simulink model "model_new"  (R2023a)
settings: Solver=VariableStepAuto  StartTime=0.0  StopTime=0.5  RelTol=1e-3
model workspace: external: MATLAB File model_new_DataFile.m (data not in the file)
values from neighbouring files (symbols this model uses):
  smiData = struct    [model_new_DataFile.m]
undefined symbols (not defined in the file or in its folder): _, ____, ____16, ____19, ____20, ____3, ____4, ____4X6X3, ____6, ____6X10X3, ____7X11X2, ______, ______1, ______2, ______3_________________________, _______1_________________________2_________________________________航发支架总装, ________, ________1, ________20__1____6, ________6, _________, __________, __________2, __________40160, __________6x16x5, ____________, ____________2, ____________3X1, ______________, ______________1X5, __________________, ___________________, ____________________20__26____4, ____________________25__25____5, __________________SULERCH, ______________A, __________A, __________B, ______A__6, _X2_4E1D6746_X0_, _X2_652F64915EA7_X0_, _X2_7535673A5B8988C5677F_X0_, _X2_8F74627F677F_X0_, _航发支架总装, _默认_sldprt, A25, a__________100, BZ, C, CONNECTOR_5MMCLOSED2PIN_MALE_1, D1, DIP_SWITCH_8PIN_VIC2_1, DYJN, EC, EE, FUS606_REF_1, GE4C, IPOS__________, LAF30, M3________ ... (+34)
libraries: sm_lib x990, nesl_utility x6, simulink x4
(part 3 of 18)

== system model_new/x__25_07_22_V1_STEP_1_RIGID/R1 ==
  Transform74 : sm_lib/Frames and Transforms/Rigid Transform  TranslationMethod=Cartesian  TranslationStandardOffset=0  TranslationStandardOffsetUnits=m  TranslationStandardAxis=+Z  TranslationCartesianOffset=smiData.RigidTransform(269).translation  TranslationCartesianOffsetUnits=mm  TranslationROffset=0  TranslationROffsetUnits=m  TranslationZOffset=0  TranslationZOffsetUnits=m  TranslationThetaOffset=0  TranslationThetaOffsetUnits=deg  RotationMethod=ArbitraryAxis  RotationAngleUnits=rad  RotationStandardAxis=+Z  RotationAngle=smiData.RigidTransform(269).angle  RotationArbitraryAxis=smiData.RigidTransform(269).axis  FollAlignAxisA=+X  BaseAlignAxisA=+Y  FollAlignAxisB=+Y  BaseAlignAxisB=+Z  RotationSequenceAxes=FollowerAxes  RotationSequence=XYX  RotationSequenceAngles=[0 0 0]  RotationSequenceAnglesUnits=deg  RotationMatrix=[1 0 0; 0 1 0; 0 0 1]  Quaternion=[1 0 0 0]
  Transform75 : sm_lib/Frames and Transforms/Rigid Transform  TranslationMethod=Cartesian  TranslationStandardOffset=0  TranslationStandardOffsetUnits=m  TranslationStandardAxis=+Z  TranslationCartesianOffset=smiData.RigidTransform(270).translation  TranslationCartesianOffsetUnits=mm  TranslationROffset=0  TranslationROffsetUnits=m  TranslationZOffset=0  TranslationZOffsetUnits=m  TranslationThetaOffset=0  TranslationThetaOffsetUnits=deg  RotationMethod=ArbitraryAxis  RotationAngleUnits=rad  RotationStandardAxis=+Z  RotationAngle=smiData.RigidTransform(270).angle  RotationArbitraryAxis=smiData.RigidTransform(270).axis  FollAlignAxisA=+X  BaseAlignAxisA=+Y  FollAlignAxisB=+Y  BaseAlignAxisB=+Z  RotationSequenceAxes=FollowerAxes  RotationSequence=XYX  RotationSequenceAngles=[0 0 0]  RotationSequenceAnglesUnits=deg  RotationMatrix=[1 0 0; 0 1 0; 0 0 1]  Quaternion=[1 0 0 0]
  Transform76 : sm_lib/Frames and Transforms/Rigid Transform  TranslationMethod=Cartesian  TranslationStandardOffset=0  TranslationStandardOffsetUnits=m  TranslationStandardAxis=+Z  TranslationCartesianOffset=smiData.RigidTransform(271).translation  TranslationCartesianOffsetUnits=mm  TranslationROffset=0  TranslationROffsetUnits=m  TranslationZOffset=0  TranslationZOffsetUnits=m  TranslationThetaOffset=0  TranslationThetaOffsetUnits=deg  RotationMethod=ArbitraryAxis  RotationAngleUnits=rad  RotationStandardAxis=+Z  RotationAngle=smiData.RigidTransform(271).angle  RotationArbitraryAxis=smiData.RigidTransform(271).axis  FollAlignAxisA=+X  BaseAlignAxisA=+Y  FollAlignAxisB=+Y  BaseAlignAxisB=+Z  RotationSequenceAxes=FollowerAxes  RotationSequence=XYX  RotationSequenceAngles=[0 0 0]  RotationSequenceAnglesUnits=deg  RotationMatrix=[1 0 0; 0 1 0; 0 0 1]  Quaternion=[1 0 0 0]
  Transform77 : sm_lib/Frames and Transforms/Rigid Transform  TranslationMethod=Cartesian  TranslationStandardOffset=0  TranslationStandardOffsetUnits=m  TranslationStandardAxis=+Z  TranslationCartesianOffset=smiData.RigidTransform(272).translation  TranslationCartesianOffsetUnits=mm  TranslationROffset=0  TranslationROffsetUnits=m  TranslationZOffset=0  TranslationZOffsetUnits=m  TranslationThetaOffset=0  TranslationThetaOffsetUnits=deg  RotationMethod=ArbitraryAxis  RotationAngleUnits=rad  RotationStandardAxis=+Z  RotationAngle=smiData.RigidTransform(272).angle  RotationArbitraryAxis=smiData.RigidTransform(272).axis  FollAlignAxisA=+X  BaseAlignAxisA=+Y  FollAlignAxisB=+Y  BaseAlignAxisB=+Z  RotationSequenceAxes=FollowerAxes  RotationSequence=XYX  RotationSequenceAngles=[0 0 0]  RotationSequenceAnglesUnits=deg  RotationMatrix=[1 0 0; 0 1 0; 0 0 1]  Quaternion=[1 0 0 0]
  Transform78 : sm_lib/Frames and Transforms/Rigid Transform  TranslationMethod=Cartesian  TranslationStandardOffset=0  TranslationStandardOffsetUnits=m  TranslationStandardAxis=+Z  TranslationCartesianOffset=smiData.RigidTransform(273).translation  TranslationCartesianOffsetUnits=mm  TranslationROffset=0  TranslationROffsetUnits=m  TranslationZOffset=0  TranslationZOffsetUnits=m  TranslationThetaOffset=0  TranslationThetaOffsetUnits=deg  RotationMethod=ArbitraryAxis  RotationAngleUnits=rad  RotationStandardAxis=+Z  RotationAngle=smiData.RigidTransform(273).angle  RotationArbitraryAxis=smiData.RigidTransform(273).axis  FollAlignAxisA=+X  BaseAlignAxisA=+Y  FollAlignAxisB=+Y  BaseAlignAxisB=+Z  RotationSequenceAxes=FollowerAxes  RotationSequence=XYX  RotationSequenceAngles=[0 0 0]  RotationSequenceAnglesUnits=deg  RotationMatrix=[1 0 0; 0 1 0; 0 0 1]  Quaternion=[1 0 0 0]
  x1_3U_STEP_1_RIGID : Subsystem
  x1_3_4X6X3_STEP_1_RIGID1 : Subsystem
  x1_3_4X6X3_STEP_2_RIGID1 : Subsystem
  Conn1 : PMIOPort  Side=Right
  Conn2 : PMIOPort  Port=2  Side=Left
  connections:
  Transform76/RConn1 -- x1_3_4X6X3_STEP_1_RIGID1/LConn1
  Transform76/LConn1 -- Transform77/LConn1 -- Transform78/RConn1 -- Transform74/LConn1 -- Transform75/LConn1
  Transform75/RConn1 -- x1_3_4X6X3_STEP_2_RIGID1/LConn1
  Transform74/RConn1 -- x1_3U_STEP_1_RIGID/LConn1
  Transform77/RConn1 -- Conn1/RConn1
  Transform78/LConn1 -- Conn2/RConn1

== system model_new/x__25_07_22_V1_STEP_1_RIGID/R2 ==
  ReferenceFrame : sm_lib/Frames and Transforms/Reference Frame
  Transform74 : sm_lib/Frames and Transforms/Rigid Transform  TranslationMethod=Cartesian  TranslationStandardOffset=0  TranslationStandardOffsetUnits=m  TranslationStandardAxis=+Z  TranslationCartesianOffset=smiData.RigidTransform(331).translation  TranslationCartesianOffsetUnits=mm  TranslationROffset=0  TranslationROffsetUnits=m  TranslationZOffset=0  TranslationZOffsetUnits=m  TranslationThetaOffset=0  TranslationThetaOffsetUnits=deg  RotationMethod=ArbitraryAxis  RotationAngleUnits=rad  RotationStandardAxis=+Z  RotationAngle=smiData.RigidTransform(331).angle  RotationArbitraryAxis=smiData.RigidTransform(331).axis  FollAlignAxisA=+X  BaseAlignAxisA=+Y  FollAlignAxisB=+Y  BaseAlignAxisB=+Z  RotationSequenceAxes=FollowerAxes  RotationSequence=XYX  RotationSequenceAngles=[0 0 0]  RotationSequenceAnglesUnits=deg  RotationMatrix=[1 0 0; 0 1 0; 0 0 1]  Quaternion=[1 0 0 0]
  Transform75 : sm_lib/Frames and Transforms/Rigid Transform  TranslationMethod=Cartesian  TranslationStandardOffset=0  TranslationStandardOffsetUnits=m  TranslationStandardAxis=+Z  TranslationCartesianOffset=smiData.RigidTransform(332).translation  TranslationCartesianOffsetUnits=mm  TranslationROffset=0  TranslationROffsetUnits=m  TranslationZOffset=0  TranslationZOffsetUnits=m  TranslationThetaOffset=0  TranslationThetaOffsetUnits=deg  RotationMethod=ArbitraryAxis  RotationAngleUnits=rad  RotationStandardAxis=+Z  RotationAngle=smiData.RigidTransform(332).angle  RotationArbitraryAxis=smiData.RigidTransform(332).axis  FollAlignAxisA=+X  BaseAlignAxisA=+Y  FollAlignAxisB=+Y  BaseAlignAxisB=+Z  RotationSequenceAxes=FollowerAxes  RotationSequence=XYX  RotationSequenceAngles=[0 0 0]  RotationSequenceAnglesUnits=deg  RotationMatrix=[1 0 0; 0 1 0; 0 0 1]  Quaternion=[1 0 0 0]
  Transform76 : sm_lib/Frames and Transforms/Rigid Transform  TranslationMethod=Cartesian  TranslationStandardOffset=0  TranslationStandardOffsetUnits=m  TranslationStandardAxis=+Z  TranslationCartesianOffset=smiData.RigidTransform(333).translation  TranslationCartesianOffsetUnits=mm  TranslationROffset=0  TranslationROffsetUnits=m  TranslationZOffset=0  TranslationZOffsetUnits=m  TranslationThetaOffset=0  TranslationThetaOffsetUnits=deg  RotationMethod=ArbitraryAxis  RotationAngleUnits=rad  RotationStandardAxis=+Z  RotationAngle=smiData.RigidTransform(333).angle  RotationArbitraryAxis=smiData.RigidTransform(333).axis  FollAlignAxisA=+X  BaseAlignAxisA=+Y  FollAlignAxisB=+Y  BaseAlignAxisB=+Z  RotationSequenceAxes=FollowerAxes  RotationSequence=XYX  RotationSequenceAngles=[0 0 0]  RotationSequenceAnglesUnits=deg  RotationMatrix=[1 0 0; 0 1 0; 0 0 1]  Quaternion=[1 0 0 0]
  Transform77 : sm_lib/Frames and Transforms/Rigid Transform  TranslationMethod=Cartesian  TranslationStandardOffset=0  TranslationStandardOffsetUnits=m  TranslationStandardAxis=+Z  TranslationCartesianOffset=smiData.RigidTransform(334).translation  TranslationCartesianOffsetUnits=mm  TranslationROffset=0  TranslationROffsetUnits=m  TranslationZOffset=0  TranslationZOffsetUnits=m  TranslationThetaOffset=0  TranslationThetaOffsetUnits=deg  RotationMethod=ArbitraryAxis  RotationAngleUnits=rad  RotationStandardAxis=+Z  RotationAngle=smiData.RigidTransform(334).angle  RotationArbitraryAxis=smiData.RigidTransform(334).axis  FollAlignAxisA=+X  BaseAlignAxisA=+Y  FollAlignAxisB=+Y  BaseAlignAxisB=+Z  RotationSequenceAxes=FollowerAxes  RotationSequence=XYX  RotationSequenceAngles=[0 0 0]  RotationSequenceAnglesUnits=deg  RotationMatrix=[1 0 0; 0 1 0; 0 0 1]  Quaternion=[1 0 0 0]
  Transform78 : sm_lib/Frames and Transforms/Rigid Transform  TranslationMethod=Cartesian  TranslationStandardOffset=0  TranslationStandardOffsetUnits=m  TranslationStandardAxis=+Z  TranslationCartesianOffset=smiData.RigidTransform(335).translation  TranslationCartesianOffsetUnits=mm  TranslationROffset=0  TranslationROffsetUnits=m  TranslationZOffset=0  TranslationZOffsetUnits=m  TranslationThetaOffset=0  TranslationThetaOffsetUnits=deg  RotationMethod=ArbitraryAxis  RotationAngleUnits=rad  RotationStandardAxis=+Z  RotationAngle=smiData.RigidTransform(335).angle  RotationArbitraryAxis=smiData.RigidTransform(335).axis  FollAlignAxisA=+X  BaseAlignAxisA=+Y  FollAlignAxisB=+Y  BaseAlignAxisB=+Z  RotationSequenceAxes=FollowerAxes  RotationSequence=XYX  RotationSequenceAngles=[0 0 0]  RotationSequenceAnglesUnits=deg  RotationMatrix=[1 0 0; 0 1 0; 0 0 1]  Quaternion=[1 0 0 0]
  x1_3U_STEP_1_RIGID : Subsystem
  x1_3_4X6X3_STEP_1_RIGID1 : Subsystem
  x1_3_4X6X3_STEP_2_RIGID1 : Subsystem
  Conn1 : PMIOPort  Side=Left
  Conn2 : PMIOPort  Port=2  Side=Right
  connections:
  Transform78/LConn1 -- Conn1/RConn1
  Transform77/RConn1 -- x1_3U_STEP_1_RIGID/LConn1
  Transform76/LConn1 -- Transform77/LConn1 -- ReferenceFrame/RConn1 -- Transform78/RConn1 -- Transform74/LConn1 -- Transform75/LConn1
  Transform74/RConn1 -- x1_3_4X6X3_STEP_2_RIGID1/LConn1
  Transform76/RConn1 -- x1_3_4X6X3_STEP_1_RIGID1/LConn1
  Transform75/RConn1 -- Conn2/RConn1

== system model_new/x__25_07_22_V1_STEP_1_RIGID/R3 ==
  ReferenceFrame : sm_lib/Frames and Transforms/Reference Frame
  Transform1 : sm_lib/Frames and Transforms/Rigid Transform  TranslationMethod=StandardAxis  TranslationStandardOffset=15  TranslationStandardOffsetUnits=mm  TranslationStandardAxis=-Y  TranslationCartesianOffset=smiData.RigidTransform(335).translation  TranslationCartesianOffsetUnits=mm  TranslationROffset=0  TranslationROffsetUnits=m  TranslationZOffset=0  TranslationZOffsetUnits=m  TranslationThetaOffset=0  TranslationThetaOffsetUnits=deg  RotationMethod=None  RotationAngleUnits=rad  RotationStandardAxis=+Z  RotationAngle=smiData.RigidTransform(335).angle  RotationArbitraryAxis=smiData.RigidTransform(335).axis  FollAlignAxisA=+X  BaseAlignAxisA=+Y  FollAlignAxisB=+Y  BaseAlignAxisB=+Z  RotationSequenceAxes=FollowerAxes  RotationSequence=XYX  RotationSequenceAngles=[0 0 0]  RotationSequenceAnglesUnits=deg  RotationMatrix=[1 0 0; 0 1 0; 0 0 1]  Quaternion=[1 0 0 0]
  Transform74 : sm_lib/Frames and Transforms/Rigid Transform  TranslationMethod=Cartesian  TranslationStandardOffset=0  TranslationStandardOffsetUnits=m  TranslationStandardAxis=+Z  TranslationCartesianOffset=smiData.RigidTransform(331).translation  TranslationCartesianOffsetUnits=mm  TranslationROffset=0  TranslationROffsetUnits=m  TranslationZOffset=0  TranslationZOffsetUnits=m  TranslationThetaOffset=0  TranslationThetaOffsetUnits=deg  RotationMethod=ArbitraryAxis  RotationAngleUnits=rad  RotationStandardAxis=+Z  RotationAngle=smiData.RigidTransform(331).angle  RotationArbitraryAxis=smiData.RigidTransform(331).axis  FollAlignAxisA=+X  BaseAlignAxisA=+Y  FollAlignAxisB=+Y  BaseAlignAxisB=+Z  RotationSequenceAxes=FollowerAxes  RotationSequence=XYX  RotationSequenceAngles=[0 0 0]  RotationSequenceAnglesUnits=deg  RotationMatrix=[1 0 0; 0 1 0; 0 0 1]  Quaternion=[1 0 0 0]
  Transform75 : sm_lib/Frames and Transforms/Rigid Transform  TranslationMethod=Cartesian  TranslationStandardOffset=0  TranslationStandardOffsetUnits=m  TranslationStandardAxis=+Z  TranslationCartesianOffset=smiData.RigidTransform(332).translation  TranslationCartesianOffsetUnits=mm  TranslationROffset=0  TranslationROffsetUnits=m  TranslationZOffset=0  TranslationZOffsetUnits=m  TranslationThetaOffset=0  TranslationThetaOffsetUnits=deg  RotationMethod=ArbitraryAxis  RotationAngleUnits=rad  RotationStandardAxis=+Z  RotationAngle=smiData.RigidTransform(332).angle  RotationArbitraryAxis=smiData.RigidTransform(332).axis  FollAlignAxisA=+X  BaseAlignAxisA=+Y  FollAlignAxisB=+Y  BaseAlignAxisB=+Z  RotationSequenceAxes=FollowerAxes  RotationSequence=XYX  RotationSequenceAngles=[0 0 0]  RotationSequenceAnglesUnits=deg  RotationMatrix=[1 0 0; 0 1 0; 0 0 1]  Quaternion=[1 0 0 0]
  Transform76 : sm_lib/Frames and Transforms/Rigid Transform  TranslationMethod=Cartesian  TranslationStandardOffset=0  TranslationStandardOffsetUnits=m  TranslationStandardAxis=+Z  TranslationCartesianOffset=smiData.RigidTransform(333).translation  TranslationCartesianOffsetUnits=mm  TranslationROffset=0  TranslationROffsetUnits=m  TranslationZOffset=0  TranslationZOffsetUnits=m  TranslationThetaOffset=0  TranslationThetaOffsetUnits=deg  RotationMethod=ArbitraryAxis  RotationAngleUnits=rad  RotationStandardAxis=+Z  RotationAngle=smiData.RigidTransform(333).angle  RotationArbitraryAxis=smiData.RigidTransform(333).axis  FollAlignAxisA=+X  BaseAlignAxisA=+Y  FollAlignAxisB=+Y  BaseAlignAxisB=+Z  RotationSequenceAxes=FollowerAxes  RotationSequence=XYX  RotationSequenceAngles=[0 0 0]  RotationSequenceAnglesUnits=deg  RotationMatrix=[1 0 0; 0 1 0; 0 0 1]  Quaternion=[1 0 0 0]
  Transform77 : sm_lib/Frames and Transforms/Rigid Transform  TranslationMethod=Cartesian  TranslationStandardOffset=0  TranslationStandardOffsetUnits=m  TranslationStandardAxis=+Z  TranslationCartesianOffset=smiData.RigidTransform(334).translation  TranslationCartesianOffsetUnits=mm  TranslationROffset=0  TranslationROffsetUnits=m  TranslationZOffset=0  TranslationZOffsetUnits=m  TranslationThetaOffset=0  TranslationThetaOffsetUnits=deg  RotationMethod=ArbitraryAxis  RotationAngleUnits=rad  RotationStandardAxis=+Z  RotationAngle=smiData.RigidTransform(334).angle  RotationArbitraryAxis=smiData.RigidTransform(334).axis  FollAlignAxisA=+X  BaseAlignAxisA=+Y  FollAlignAxisB=+Y  BaseAlignAxisB=+Z  RotationSequenceAxes=FollowerAxes  RotationSequence=XYX  RotationSequenceAngles=[0 0 0]  RotationSequenceAnglesUnits=deg  RotationMatrix=[1 0 0; 0 1 0; 0 0 1]  Quaternion=[1 0 0 0]
  Transform78 : sm_lib/Frames and Transforms/Rigid Transform  TranslationMethod=Cartesian  TranslationStandardOffset=0  TranslationStandardOffsetUnits=m  TranslationStandardAxis=+Z  TranslationCartesianOffset=smiData.RigidTransform(335).translation  TranslationCartesianOffsetUnits=mm  TranslationROffset=0  TranslationROffsetUnits=m  TranslationZOffset=0  TranslationZOffsetUnits=m  TranslationThetaOffset=0  TranslationThetaOffsetUnits=deg  RotationMethod=ArbitraryAxis  RotationAngleUnits=rad  RotationStandardAxis=+Z  RotationAngle=smiData.RigidTransform(335).angle  RotationArbitraryAxis=smiData.RigidTransform(335).axis  FollAlignAxisA=+X  BaseAlignAxisA=+Y  FollAlignAxisB=+Y  BaseAlignAxisB=+Z  RotationSequenceAxes=FollowerAxes  RotationSequence=XYX  RotationSequenceAngles=[0 0 0]  RotationSequenceAnglesUnits=deg  RotationMatrix=[1 0 0; 0 1 0; 0 0 1]  Quaternion=[1 0 0 0]
  x1_3U_STEP_1_RIGID : Subsystem
  x1_3_4X6X3_STEP_1_RIGID1 : Subsystem
  x1_3_4X6X3_STEP_2_RIGID1 : Subsystem
  Conn1 : PMIOPort  Side=Left
  Conn2 : PMIOPort  Port=2  Side=Right
  connections:
  Transform1/LConn1 -- Transform78/RConn1
  Transform77/RConn1 -- x1_3U_STEP_1_RIGID/LConn1
  Transform78/LConn1 -- Conn1/RConn1
  Transform76/RConn1 -- x1_3_4X6X3_STEP_1_RIGID1/LConn1
  Transform74/RConn1 -- x1_3_4X6X3_STEP_2_RIGID1/LConn1
  Transform75/RConn1 -- Conn2/RConn1
  Transform76/LConn1 -- Transform77/LConn1 -- ReferenceFrame/RConn1 -- Transform1/RConn1 -- Transform74/LConn1 -- Transform75/LConn1

== system model_new/x__25_07_22_V1_STEP_1_RIGID/R4 ==
  ReferenceFrame : sm_lib/Frames and Transforms/Reference Frame
  Transform74 : sm_lib/Frames and Transforms/Rigid Transform  TranslationMethod=Cartesian  TranslationStandardOffset=0  TranslationStandardOffsetUnits=m  TranslationStandardAxis=+Z  TranslationCartesianOffset=smiData.RigidTransform(311).translation  TranslationCartesianOffsetUnits=mm  TranslationROffset=0  TranslationROffsetUnits=m  TranslationZOffset=0  TranslationZOffsetUnits=m  TranslationThetaOffset=0  TranslationThetaOffsetUnits=deg  RotationMethod=ArbitraryAxis  RotationAngleUnits=rad  RotationStandardAxis=+Z  RotationAngle=smiData.RigidTransform(311).angle  RotationArbitraryAxis=smiData.RigidTransform(311).axis  FollAlignAxisA=+X  BaseAlignAxisA=+Y  FollAlignAxisB=+Y  BaseAlignAxisB=+Z  RotationSequenceAxes=FollowerAxes  RotationSequence=XYX  RotationSequenceAngles=[0 0 0]  RotationSequenceAnglesUnits=deg  RotationMatrix=[1 0 0; 0 1 0; 0 0 1]  Quaternion=[1 0 0 0]
  Transform75 : sm_lib/Frames and Transforms/Rigid Transform  TranslationMethod=Cartesian  TranslationStandardOffset=0  TranslationStandardOffsetUnits=m  TranslationStandardAxis=+Z  TranslationCartesianOffset=smiData.RigidTransform(312).translation  TranslationCartesianOffsetUnits=mm  TranslationROffset=0  TranslationROffsetUnits=m  TranslationZOffset=0  TranslationZOffsetUnits=m  TranslationThetaOffset=0  TranslationThetaOffsetUnits=deg  RotationMethod=ArbitraryAxis  RotationAngleUnits=rad  RotationStandardAxis=+Z  RotationAngle=smiData.RigidTransform(312).angle  RotationArbitraryAxis=smiData.RigidTransform(312).axis  FollAlignAxisA=+X  BaseAlignAxisA=+Y  FollAlignAxisB=+Y  BaseAlignAxisB=+Z  RotationSequenceAxes=FollowerAxes  RotationSequence=XYX  RotationSequenceAngles=[0 0 0]  RotationSequenceAnglesUnits=deg  RotationMatrix=[1 0 0; 0 1 0; 0 0 1]  Quaternion=[1 0 0 0]
  Transform76 : sm_lib/Frames and Transforms/Rigid Transform  TranslationMethod=Cartesian  TranslationStandardOffset=0  TranslationStandardOffsetUnits=m  TranslationStandardAxis=+Z  TranslationCartesianOffset=smiData.RigidTransform(313).translation  TranslationCartesianOffsetUnits=mm  TranslationROffset=0  TranslationROffsetUnits=m  TranslationZOffset=0  TranslationZOffsetUnits=m  TranslationThetaOffset=0  TranslationThetaOffsetUnits=deg  RotationMethod=ArbitraryAxis  RotationAngleUnits=rad  RotationStandardAxis=+Z  RotationAngle=smiData.RigidTransform(313).angle  RotationArbitraryAxis=smiData.RigidTransform(313).axis  FollAlignAxisA=+X  BaseAlignAxisA=+Y  FollAlignAxisB=+Y  BaseAlignAxisB=+Z  RotationSequenceAxes=FollowerAxes  RotationSequence=XYX  RotationSequenceAngles=[0 0 0]  RotationSequenceAnglesUnits=deg  RotationMatrix=[1 0 0; 0 1 0; 0 0 1]  Quaternion=[1 0 0 0]
  Transform77 : sm_lib/Frames and Transforms/Rigid Transform  TranslationMethod=Cartesian  TranslationStandardOffset=0  TranslationStandardOffsetUnits=m  TranslationStandardAxis=+Z  TranslationCartesianOffset=smiData.RigidTransform(314).translation  TranslationCartesianOffsetUnits=mm  TranslationROffset=0  TranslationROffsetUnits=m  TranslationZOffset=0  TranslationZOffsetUnits=m  TranslationThetaOffset=0  TranslationThetaOffsetUnits=deg  RotationMethod=ArbitraryAxis  RotationAngleUnits=rad  RotationStandardAxis=+Z  RotationAngle=smiData.RigidTransform(314).angle  RotationArbitraryAxis=smiData.RigidTransform(314).axis  FollAlignAxisA=+X  BaseAlignAxisA=+Y  FollAlignAxisB=+Y  BaseAlignAxisB=+Z  RotationSequenceAxes=FollowerAxes  RotationSequence=XYX  RotationSequenceAngles=[0 0 0]  RotationSequenceAnglesUnits=deg  RotationMatrix=[1 0 0; 0 1 0; 0 0 1]  Quaternion=[1 0 0 0]
  Transform78 : sm_lib/Frames and Transforms/Rigid Transform  TranslationMethod=Cartesian  TranslationStandardOffset=0  TranslationStandardOffsetUnits=m  TranslationStandardAxis=+Z  TranslationCartesianOffset=smiData.RigidTransform(315).translation  TranslationCartesianOffsetUnits=mm  TranslationROffset=0  TranslationROffsetUnits=m  TranslationZOffset=0  TranslationZOffsetUnits=m  TranslationThetaOffset=0  TranslationThetaOffsetUnits=deg  RotationMethod=ArbitraryAxis  RotationAngleUnits=rad  RotationStandardAxis=+Z  RotationAngle=smiData.RigidTransform(315).angle  RotationArbitraryAxis=smiData.RigidTransform(315).axis  FollAlignAxisA=+X  BaseAlignAxisA=+Y  FollAlignAxisB=+Y  BaseAlignAxisB=+Z  RotationSequenceAxes=FollowerAxes  RotationSequence=XYX  RotationSequenceAngles=[0 0 0]  RotationSequenceAnglesUnits=deg  RotationMatrix=[1 0 0; 0 1 0; 0 0 1]  Quaternion=[1 0 0 0]
  x1_3U_STEP_1_RIGID : Subsystem
  x1_3_4X6X3_STEP_1_RIGID1 : Subsystem
  x1_3_4X6X3_STEP_2_RIGID1 : Subsystem
  Conn1 : PMIOPort  Side=Left
  Conn2 : PMIOPort  Port=2  Side=Right
  connections:
  Transform76/LConn1 -- Transform77/LConn1 -- ReferenceFrame/RConn1 -- Transform78/RConn1 -- Transform74/LConn1 -- Transform75/LConn1
  Transform77/RConn1 -- x1_3U_STEP_1_RIGID/LConn1
  Transform75/RConn1 -- x1_3_4X6X3_STEP_2_RIGID1/LConn1
  Conn1/RConn1 -- Transform78/LConn1
  Transform74/RConn1 -- x1_3_4X6X3_STEP_1_RIGID1/LConn1
  Transform76/RConn1 -- Conn2/RConn1

== system model_new/x__25_07_22_V1_STEP_1_RIGID/Subsystem ==
  C_MPU10_20_38_30_STEP_1_RIGID : Subsystem
  ReferenceFrame : sm_lib/Frames and Transforms/Reference Frame
  Transform : sm_lib/Frames and Transforms/Rigid Transform  TranslationMethod=Cartesian  TranslationStandardOffset=0  TranslationStandardOffsetUnits=m  TranslationStandardAxis=+Z  TranslationCartesianOffset=smiData.RigidTransform(222).translation  TranslationCartesianOffsetUnits=mm  TranslationROffset=0  TranslationROffsetUnits=m  TranslationZOffset=0  TranslationZOffsetUnits=m  TranslationThetaOffset=0  TranslationThetaOffsetUnits=deg  RotationMethod=ArbitraryAxis  RotationAngleUnits=rad  RotationStandardAxis=+Z  RotationAngle=smiData.RigidTransform(222).angle  RotationArbitraryAxis=smiData.RigidTransform(222).axis  FollAlignAxisA=+X  BaseAlignAxisA=+Y  FollAlignAxisB=+Y  BaseAlignAxisB=+Z  RotationSequenceAxes=FollowerAxes  RotationSequence=XYX  RotationSequenceAngles=[0 0 0]  RotationSequenceAnglesUnits=deg  RotationMatrix=[1 0 0; 0 1 0; 0 0 1]  Quaternion=[1 0 0 0]
  Transformc : sm_lib/Frames and Transforms/Rigid Transform  TranslationMethod=Cartesian  TranslationStandardOffset=0  TranslationStandardOffsetUnits=m  TranslationStandardAxis=+Z  TranslationCartesianOffset=smiData.RigidTransform(223).translation  TranslationCartesianOffsetUnits=mm  TranslationROffset=0  TranslationROffsetUnits=m  TranslationZOffset=0  TranslationZOffsetUnits=m  TranslationThetaOffset=0  TranslationThetaOffsetUnits=deg  RotationMethod=ArbitraryAxis  RotationAngleUnits=rad  RotationStandardAxis=+Z  RotationAngle=smiData.RigidTransform(223).angle  RotationArbitraryAxis=smiData.RigidTransform(223).axis  FollAlignAxisA=+X  BaseAlignAxisA=+Y  FollAlignAxisB=+Y  BaseAlignAxisB=+Z  RotationSequenceAxes=FollowerAxes  RotationSequence=XYX  RotationSequenceAngles=[0 0 0]  RotationSequenceAnglesUnits=deg  RotationMatrix=[1 0 0; 0 1 0; 0 0 1]  Quaternion=[1 0 0 0]
  Transformd : sm_lib/Frames and Transforms/Rigid Transform  TranslationMethod=Cartesian  TranslationStandardOffset=0  TranslationStandardOffsetUnits=m  TranslationStandardAxis=+Z  TranslationCartesianOffset=smiData.RigidTransform(221).translation  TranslationCartesianOffsetUnits=mm  TranslationROffset=0  TranslationROffsetUnits=m  TranslationZOffset=0  TranslationZOffsetUnits=m  TranslationThetaOffset=0  TranslationThetaOffsetUnits=deg  RotationMethod=ArbitraryAxis  RotationAngleUnits=rad  RotationStandardAxis=+Z  RotationAngle=smiData.RigidTransform(221).angle  RotationArbitraryAxis=smiData.RigidTransform(221).axis  FollAlignAxisA=+X  BaseAlignAxisA=+Y  FollAlignAxisB=+Y  BaseAlignAxisB=+Z  RotationSequenceAxes=FollowerAxes  RotationSequence=XYX  RotationSequenceAngles=[0 0 0]  RotationSequenceAnglesUnits=deg  RotationMatrix=[1 0 0; 0 1 0; 0 0 1]  Quaternion=[1 0 0 0]
  Transforme : sm_lib/Frames and Transforms/Rigid Transform  TranslationMethod=Cartesian  TranslationStandardOffset=0  TranslationStandardOffsetUnits=m  TranslationStandardAxis=+Z  TranslationCartesianOffset=smiData.RigidTransform(201).translation  TranslationCartesianOffsetUnits=mm  TranslationROffset=0  TranslationROffsetUnits=m  TranslationZOffset=0  TranslationZOffsetUnits=m  TranslationThetaOffset=0  TranslationThetaOffsetUnits=deg  RotationMethod=ArbitraryAxis  RotationAngleUnits=rad  RotationStandardAxis=+Z  RotationAngle=smiData.RigidTransform(201).angle  RotationArbitraryAxis=smiData.RigidTransform(201).axis  FollAlignAxisA=+X  BaseAlignAxisA=+Y  FollAlignAxisB=+Y  BaseAlignAxisB=+Z  RotationSequenceAxes=FollowerAxes  RotationSequence=XYX  RotationSequenceAngles=[0 0 0]  RotationSequenceAnglesUnits=deg  RotationMatrix=[1 0 0; 0 1 0; 0 0 1]  Quaternion=[1 0 0 0]
  x__25_07_22_V1_STEP_1_RIGID1 : Subsystem
  x__STEP_1_RIGID : Subsystem
  Conn1 : PMIOPort  Side=Right
  Conn2 : PMIOPort  Port=2  Side=Left
  connections:
  Transform/RConn1 -- x__STEP_1_RIGID/LConn1
  Transforme/RConn1 -- Conn1/RConn1
  Transforme/LConn1 -- Transformd/RConn1
  ReferenceFrame/RConn1 -- x__25_07_22_V1_STEP_1_RIGID1/LConn1 -- Transformd/LConn1 -- Transform/LConn1 -- Transformc/RConn1 -- C_MPU10_20_38_30_STEP_1_RIGID/LConn1
  Transformc/LConn1 -- Conn2/RConn1
